simulink library "PMSMPlant"  (R2026a)
settings: Solver=VariableStepAuto
undefined symbols (not defined in the file or in its folder): pmsmCfg
settings Model: Creator=24322  LastModifiedBy=24322

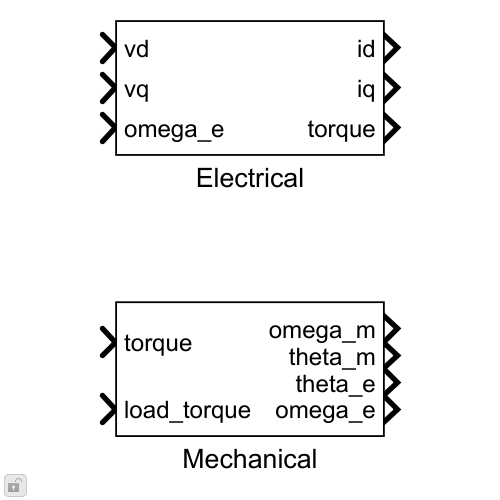
[thumbnail: Simulink's stored preview of the top-level diagram]
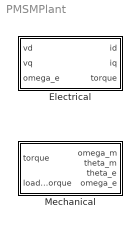
== system PMSMPlant ==
  Electrical : Subsystem
  Mechanical : Subsystem

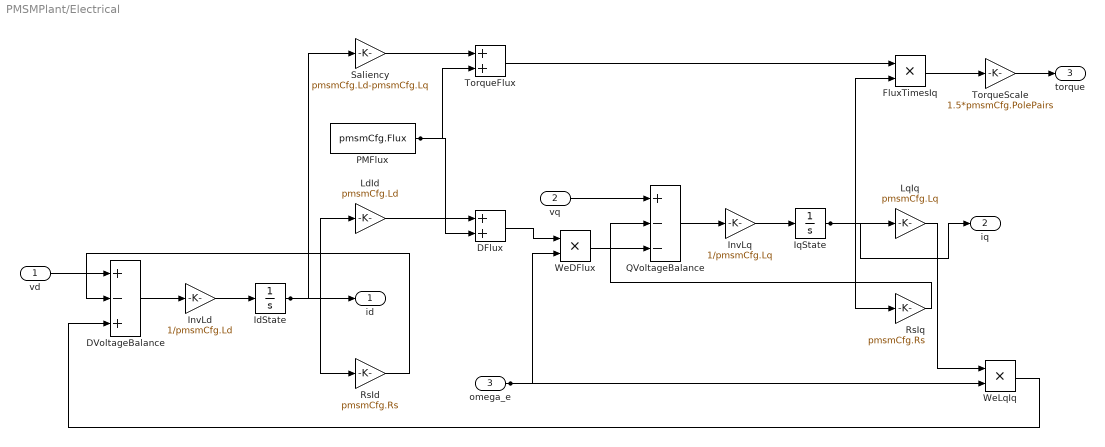
== system PMSMPlant/Electrical ==
  vd : Inport
  vq : Inport  Port=2
  omega_e : Inport  Port=3
  DFlux : Sum
  DVoltageBalance : Sum  Inputs=+-+
  FluxTimesIq : Product
  IdState : Integrator  InitialCondition=pmsmCfg.Id0
  InvLd : Gain  Gain=1/pmsmCfg.Ld
  InvLq : Gain  Gain=1/pmsmCfg.Lq
  IqState : Integrator  InitialCondition=pmsmCfg.Iq0
  LdId : Gain  Gain=pmsmCfg.Ld
  LqIq : Gain  Gain=pmsmCfg.Lq
  PMFlux : Constant  Value=pmsmCfg.Flux
  QVoltageBalance : Sum  Inputs=+--
  RsId : Gain  Gain=pmsmCfg.Rs
  RsIq : Gain  Gain=pmsmCfg.Rs
  Saliency : Gain  Gain=pmsmCfg.Ld-pmsmCfg.Lq
  TorqueFlux : Sum
  TorqueScale : Gain  Gain=1.5*pmsmCfg.PolePairs
  WeDFlux : Product
  WeLqIq : Product
  id : Outport
  iq : Outport  Port=2
  torque : Outport  Port=3
  wires:
  TorqueScale/1 -> torque/1
  FluxTimesIq/1 -> TorqueScale/1
  TorqueFlux/1 -> FluxTimesIq/1
  Saliency/1 -> TorqueFlux/1
  DFlux/1 -> WeDFlux/1
  PMFlux/1 -> DFlux/2, TorqueFlux/2
  LdId/1 -> DFlux/1
  omega_e/1 -> WeLqIq/2, WeDFlux/2
  LqIq/1 -> WeLqIq/1
  IqState/1 -> RsIq/1, iq/1, LqIq/1, FluxTimesIq/2
  IdState/1 -> RsId/1, LdId/1, Saliency/1, id/1
  InvLq/1 -> IqState/1
  QVoltageBalance/1 -> InvLq/1
  WeDFlux/1 -> QVoltageBalance/3
  RsIq/1 -> QVoltageBalance/2
  vq/1 -> QVoltageBalance/1
  InvLd/1 -> IdState/1
  DVoltageBalance/1 -> InvLd/1
  WeLqIq/1 -> DVoltageBalance/3
  RsId/1 -> DVoltageBalance/2
  vd/1 -> DVoltageBalance/1

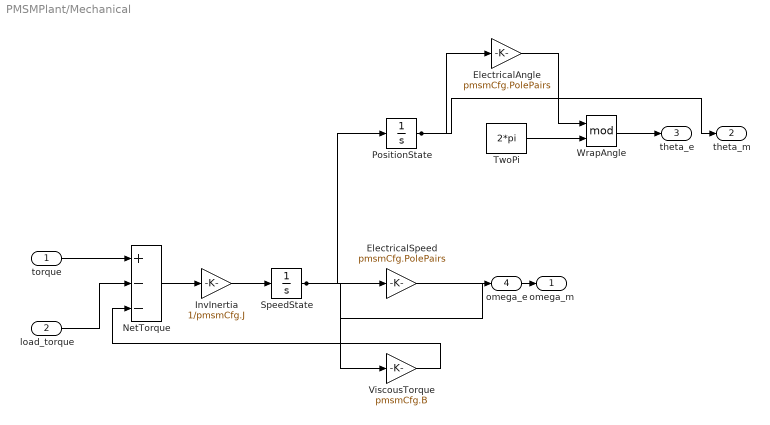
== system PMSMPlant/Mechanical ==
  torque : Inport
  load_torque : Inport  Port=2
  ElectricalAngle : Gain  Gain=pmsmCfg.PolePairs
  ElectricalSpeed : Gain  Gain=pmsmCfg.PolePairs
  InvInertia : Gain  Gain=1/pmsmCfg.J
  NetTorque : Sum  Inputs=+--
  PositionState : Integrator  InitialCondition=pmsmCfg.Position0
  SpeedState : Integrator  InitialCondition=pmsmCfg.Speed0
  TwoPi : Constant  Value=2*pi
  ViscousTorque : Gain  Gain=pmsmCfg.B
  WrapAngle : Math  Operator=mod
  omega_m : Outport
  theta_m : Outport  Port=2
  theta_e : Outport  Port=3
  omega_e : Outport  Port=4
  wires:
  ElectricalSpeed/1 -> omega_e/1
  WrapAngle/1 -> theta_e/1
  TwoPi/1 -> WrapAngle/2
  ElectricalAngle/1 -> WrapAngle/1
  PositionState/1 -> ElectricalAngle/1, theta_m/1
  SpeedState/1 -> PositionState/1, omega_m/1, ViscousTorque/1, ElectricalSpeed/1
  InvInertia/1 -> SpeedState/1
  NetTorque/1 -> InvInertia/1
  ViscousTorque/1 -> NetTorque/3
  load_torque/1 -> NetTorque/2
  torque/1 -> NetTorque/1
